simulink model "Simscape_model_Energy"  (R2026a)
settings: Solver=FixedStepAuto  StopTime=8  FixedStep=0.0001
model workspace (MATLAB code in the model file):
  | clear; clc; close all;
values from neighbouring files (symbols this model uses):
  black = partTemplate    [Parameters.m]    (also in Parameters_optimization.m = struct)
  blueBlock = partTemplate    [Parameters.m]    (also in Parameters_optimization.m = struct)
  cyan = partTemplate    [Parameters.m]    (also in Parameters_optimization.m = struct)
  g = 9.81    [Parameters.m]    (also in Parameters_optimization.m)
  greenBeam = partTemplate    [Parameters.m]    (also in Parameters_optimization.m = struct)
  greenBlock = partTemplate    [Parameters.m]    (also in Parameters_optimization.m = struct)
  grey = partTemplate    [Parameters.m]    (also in Parameters_optimization.m = struct)
  IMax = 16    [Parameters.m]    (also in Parameters_optimization.m)
  IMin = -16    [Parameters.m]    (also in Parameters_optimization.m)
  JM = 0.002    [Parameters.m]    (also in Parameters_optimization.m)
  KdA_pos = 1    [Parameters.m]    (also in Parameters_optimization.m = 5066.74)
  KdA_vel = 0    [Parameters.m]    (also in Parameters_optimization.m)
  KdB1_pos = 1    [Parameters.m]    (also in Parameters_optimization.m = 4.04669)
  KdB1_vel = 0    [Parameters.m]    (also in Parameters_optimization.m)
  KdB2_pos = 1    [Parameters.m]    (also in Parameters_optimization.m = 1.06194)
  KdB2_vel = 0    [Parameters.m]    (also in Parameters_optimization.m)
  KdG_pos = 1    [Parameters.m]    (also in Parameters_optimization.m = 1.01282)
  KdG_vel = 0    [Parameters.m]    (also in Parameters_optimization.m)
  KdH_pos = 1    [Parameters.m]    (also in Parameters_optimization.m = 16.6487)
  KdH_vel = 0    [Parameters.m]    (also in Parameters_optimization.m)
  KdI_pos = 1    [Parameters.m]    (also in Parameters_optimization.m = 2.31436)
  KdI_vel = 0    [Parameters.m]    (also in Parameters_optimization.m)
  KiA_pos = 2    [Parameters.m]    (also in Parameters_optimization.m = 1.00755)
  KiA_vel = 5    [Parameters.m]    (also in Parameters_optimization.m)
  KiB1_pos = 30    [Parameters.m]    (also in Parameters_optimization.m = 45.4381)
  KiB1_vel = 10    [Parameters.m]    (also in Parameters_optimization.m)
  KiB2_pos = 20    [Parameters.m]    (also in Parameters_optimization.m = 84.4311)
  KiB2_vel = 5    [Parameters.m]    (also in Parameters_optimization.m)
  KiG_pos = 30    [Parameters.m]    (also in Parameters_optimization.m = 81.5274)
  KiG_vel = 5    [Parameters.m]    (also in Parameters_optimization.m)
  KiH_pos = 10    [Parameters.m]    (also in Parameters_optimization.m = 20739.8)
  KiH_vel = 0    [Parameters.m]    (also in Parameters_optimization.m)
  KiI_pos = 0    [Parameters.m]    (also in Parameters_optimization.m = 1)
  KiI_vel = 0    [Parameters.m]    (also in Parameters_optimization.m)
  KmA = 1.5    [Parameters.m]    (also in Parameters_optimization.m = 1)
  KmB1 = 1.5    [Parameters.m]    (also in Parameters_optimization.m)
  KmB2 = 1.5    [Parameters.m]    (also in Parameters_optimization.m = 1)
  KmG = 0.5    [Parameters.m]    (also in Parameters_optimization.m)
  KmH = 1    [Parameters.m]    (also in Parameters_optimization.m = 0.5)
  KmI = 0.5    [Parameters.m]    (also in Parameters_optimization.m)
  KpA_pos = 150    [Parameters.m]    (also in Parameters_optimization.m = 1588.6)
  KpA_vel = 30    [Parameters.m]    (also in Parameters_optimization.m)
  KpB1_pos = 200    [Parameters.m]    (also in Parameters_optimization.m = 698393)
  KpB1_vel = 30    [Parameters.m]    (also in Parameters_optimization.m)
  KpB2_pos = 150    [Parameters.m]    (also in Parameters_optimization.m = 504375)
  KpB2_vel = 30    [Parameters.m]    (also in Parameters_optimization.m)
  KpG_pos = 100    [Parameters.m]    (also in Parameters_optimization.m = 2817.67)
  KpG_vel = 50    [Parameters.m]    (also in Parameters_optimization.m)
  KpH_pos = 100    [Parameters.m]    (also in Parameters_optimization.m = 12634.3)
  KpH_vel = 20    [Parameters.m]    (also in Parameters_optimization.m)
  KpI_pos = 50    [Parameters.m]    (also in Parameters_optimization.m = 2283.96)
  KpI_vel = 20    [Parameters.m]    (also in Parameters_optimization.m)
  LB1 = 0.8    [Parameters.m]    (also in Parameters_optimization.m)
  LB2 = 0.3    [Parameters.m]    (also in Parameters_optimization.m)
  LB3 = 0.24    [Parameters.m]    (also in Parameters_optimization.m)
  Lblack1 = 0.2    [Parameters.m]    (also in Parameters_optimization.m)
  LC1 = 0.4    [Parameters.m]    (also in Parameters_optimization.m)
  LC2 = 0.225    [Parameters.m]    (also in Parameters_optimization.m)
  LG1 = 0.3    [Parameters.m]    (also in Parameters_optimization.m)
  LG2 = 0.8    [Parameters.m]    (also in Parameters_optimization.m)
  Lgrey1 = 1.175    [Parameters.m]    (also in Parameters_optimization.m)
  lightBlue = partTemplate    [Parameters.m]    (also in Parameters_optimization.m = struct)
  LLB1 = 0.248    [Parameters.m]    (also in Parameters_optimization.m)
  LLB2 = 0.235    [Parameters.m]    (also in Parameters_optimization.m)
  LR1 = 1.05    [Parameters.m]    (also in Parameters_optimization.m)
  LW1 = 1.05    [Parameters.m]    (also in Parameters_optimization.m)
  nA = 200    [Parameters.m]    (also in Parameters_optimization.m = 100)
  nB1 = 200    [Parameters.m]    (also in Parameters_optimization.m = 100)
  nB2 = 200    [Parameters.m]    (also in Parameters_optimization.m)
  nG = 20    [Parameters.m]    (also in Parameters_optimization.m)
  nH = 100    [Parameters.m]    (also in Parameters_optimization.m = 50)
  nI = 20    [Parameters.m]    (also in Parameters_optimization.m)
  omegaFilterA_pos = 60    [Parameters.m]    (also in Parameters_optimization.m)
  omegaFilterA_vel = 60    [Parameters.m]    (also in Parameters_optimization.m)
  omegaFilterB1_pos = 60    [Parameters.m]    (also in Parameters_optimization.m)
  omegaFilterB1_vel = 60    [Parameters.m]    (also in Parameters_optimization.m)
  omegaFilterB2_pos = 60    [Parameters.m]    (also in Parameters_optimization.m)
  omegaFilterB2_vel = 60    [Parameters.m]    (also in Parameters_optimization.m)
  omegaFilterG_pos = 60    [Parameters.m]    (also in Parameters_optimization.m)
  omegaFilterG_vel = 60    [Parameters.m]    (also in Parameters_optimization.m)
  omegaFilterH_pos = 60    [Parameters.m]    (also in Parameters_optimization.m)
  omegaFilterH_vel = 60    [Parameters.m]    (also in Parameters_optimization.m)
  omegaFilterI_pos = 60    [Parameters.m]    (also in Parameters_optimization.m)
  omegaFilterI_vel = 60    [Parameters.m]    (also in Parameters_optimization.m)
  red = partTemplate    [Parameters.m]    (also in Parameters_optimization.m = struct)
  trajCoeff = coeff    [Parameters.m]    (also in Parameters_optimization.m = [2000 500 1600; Path_Planning_Robot.m)
  trajTime = t    [Parameters.m]    (also in Parameters_optimization.m = [0 2 4 6 8]; Path_Planning_Robot.m)
  w = 0.1    [Parameters.m]    (also in Parameters_optimization.m)
  white = partTemplate    [Parameters.m]    (also in Parameters_optimization.m = struct)
undefined symbols (not defined in the file or in its folder): X, Y, Z
libraries: sm_lib x102, nesl_utility x58, simulink x1
(part 2 of 4)

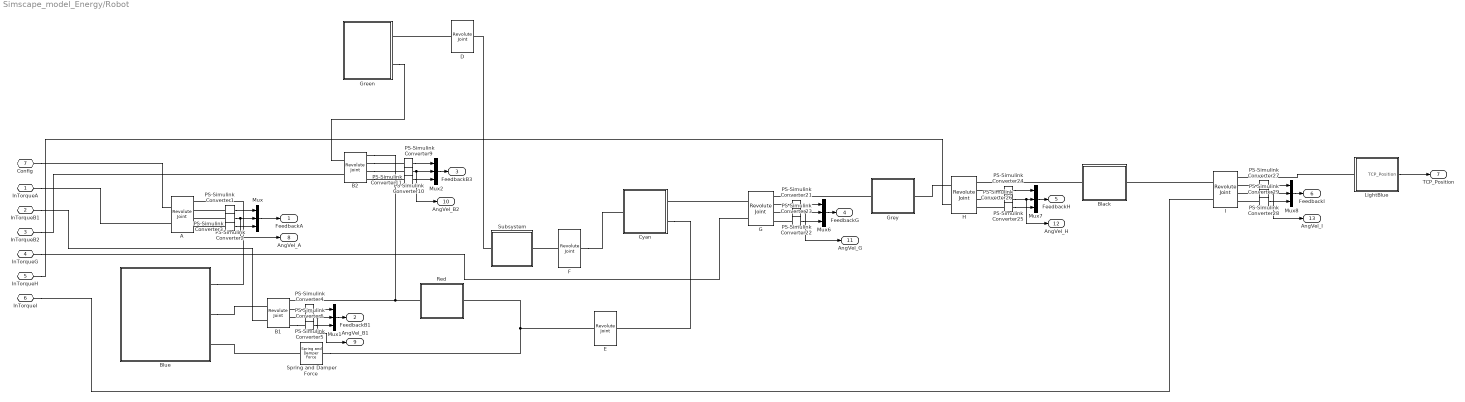
== system Simscape_model_Energy/Robot ==
  A : sm_lib/Joints/Revolute Joint  JointMode=Normal  CompositeWrenchDir=FollowerOnBase  CompositeWrenchFrame=BaseFrame  SenseConstraintForce=off  SenseConstraintTorque=off  SenseTotalForce=off  SenseTotalTorque=off  PositionTargetSpecify=on  PositionTargetPriority=High  PositionTargetValue=A0  PositionTargetValueUnits=rad  VelocityTargetSpecify=off  VelocityTargetPriority=High  VelocityTargetValue=0  VelocityTargetValueUnits=deg/s  EquilibriumPosition=0  EquilibriumPositionUnits=deg  SpringStiffness=0  SpringStiffnessUnits=N*m/deg  DampingCoefficient=0  DampingCoefficientUnits=N*m/(deg/s)  LowerLimitSpecify=off  LowerLimitBound=-90  LowerLimitBoundUnits=deg  LowerLimitStiffness=1e4  LowerLimitStiffnessUnits=N*m/deg  LowerLimitDamping=10  LowerLimitDampingUnits=N*m/(deg/s)  LowerLimitTransitionRegionWidth=0.1  LowerLimitTransitionRegionWidthUnits=deg  UpperLimitSpecify=off  UpperLimitBound=90  UpperLimitBoundUnits=deg  UpperLimitStiffness=1e4  UpperLimitStiffnessUnits=N*m/deg  UpperLimitDamping=10  UpperLimitDampingUnits=N*m/(deg/s)  UpperLimitTransitionRegionWidth=0.1  UpperLimitTransitionRegionWidthUnits=deg  TorqueActuationMode=InputTorque  MotionActuationMode=ComputedMotion  SensePosition=on  SenseVelocity=on  SenseAcceleration=on  SenseTorqueForce=off  SenseLowerLimitTorqueForce=off  SenseUpperLimitTorqueForce=off
  B1 : sm_lib/Joints/Revolute Joint  JointMode=Normal  CompositeWrenchDir=FollowerOnBase  CompositeWrenchFrame=BaseFrame  SenseConstraintForce=off  SenseConstraintTorque=off  SenseTotalForce=off  SenseTotalTorque=off  PositionTargetSpecify=on  PositionTargetPriority=High  PositionTargetValue=B10  PositionTargetValueUnits=rad  VelocityTargetSpecify=off  VelocityTargetPriority=High  VelocityTargetValue=0  VelocityTargetValueUnits=deg/s  EquilibriumPosition=0  EquilibriumPositionUnits=deg  SpringStiffness=0  SpringStiffnessUnits=N*m/deg  DampingCoefficient=0  DampingCoefficientUnits=N*m/(deg/s)  LowerLimitSpecify=on  LowerLimitBound=-80  LowerLimitBoundUnits=deg  LowerLimitStiffness=1e6  LowerLimitStiffnessUnits=N*m/deg  LowerLimitDamping=1000  LowerLimitDampingUnits=N*m/(deg/s)  LowerLimitTransitionRegionWidth=0.1  LowerLimitTransitionRegionWidthUnits=deg  UpperLimitSpecify=on  UpperLimitBound=80  UpperLimitBoundUnits=deg  UpperLimitStiffness=1e6  UpperLimitStiffnessUnits=N*m/deg  UpperLimitDamping=1000  UpperLimitDampingUnits=N*m/(deg/s)  UpperLimitTransitionRegionWidth=0.1  UpperLimitTransitionRegionWidthUnits=deg  TorqueActuationMode=InputTorque  MotionActuationMode=ComputedMotion  SensePosition=on  SenseVelocity=on  SenseAcceleration=on  SenseTorqueForce=off  SenseLowerLimitTorqueForce=off  SenseUpperLimitTorqueForce=off
  B2 : sm_lib/Joints/Revolute Joint  JointMode=Normal  CompositeWrenchDir=FollowerOnBase  CompositeWrenchFrame=BaseFrame  SenseConstraintForce=off  SenseConstraintTorque=off  SenseTotalForce=off  SenseTotalTorque=off  PositionTargetSpecify=on  PositionTargetPriority=High  PositionTargetValue=B20  PositionTargetValueUnits=rad  VelocityTargetSpecify=off  VelocityTargetPriority=High  VelocityTargetValue=0  VelocityTargetValueUnits=deg/s  EquilibriumPosition=0  EquilibriumPositionUnits=deg  SpringStiffness=0  SpringStiffnessUnits=N*m/deg  DampingCoefficient=0  DampingCoefficientUnits=N*m/(deg/s)  LowerLimitSpecify=off  LowerLimitBound=-90  LowerLimitBoundUnits=deg  LowerLimitStiffness=1e4  LowerLimitStiffnessUnits=N*m/deg  LowerLimitDamping=10  LowerLimitDampingUnits=N*m/(deg/s)  LowerLimitTransitionRegionWidth=0.1  LowerLimitTransitionRegionWidthUnits=deg  UpperLimitSpecify=off  UpperLimitBound=90  UpperLimitBoundUnits=deg  UpperLimitStiffness=1e4  UpperLimitStiffnessUnits=N*m/deg  UpperLimitDamping=10  UpperLimitDampingUnits=N*m/(deg/s)  UpperLimitTransitionRegionWidth=0.1  UpperLimitTransitionRegionWidthUnits=deg  TorqueActuationMode=InputTorque  MotionActuationMode=ComputedMotion  SensePosition=on  SenseVelocity=on  SenseAcceleration=on  SenseTorqueForce=off  SenseLowerLimitTorqueForce=off  SenseUpperLimitTorqueForce=off
  Black : Subsystem
  Blue : Subsystem
  Cyan : Subsystem
  D : sm_lib/Joints/Revolute Joint  JointMode=Normal  CompositeWrenchDir=FollowerOnBase  CompositeWrenchFrame=BaseFrame  SenseConstraintForce=off  SenseConstraintTorque=off  SenseTotalForce=off  SenseTotalTorque=off  PositionTargetSpecify=off  PositionTargetPriority=High  PositionTargetValue=0  PositionTargetValueUnits=deg  VelocityTargetSpecify=off  VelocityTargetPriority=High  VelocityTargetValue=0  VelocityTargetValueUnits=deg/s  EquilibriumPosition=0  EquilibriumPositionUnits=deg  SpringStiffness=0  SpringStiffnessUnits=N*m/deg  DampingCoefficient=0  DampingCoefficientUnits=N*m/(deg/s)  LowerLimitSpecify=off  LowerLimitBound=-90  LowerLimitBoundUnits=deg  LowerLimitStiffness=1e4  LowerLimitStiffnessUnits=N*m/deg  LowerLimitDamping=10  LowerLimitDampingUnits=N*m/(deg/s)  LowerLimitTransitionRegionWidth=0.1  LowerLimitTransitionRegionWidthUnits=deg  UpperLimitSpecify=off  UpperLimitBound=90  UpperLimitBoundUnits=deg  UpperLimitStiffness=1e4  UpperLimitStiffnessUnits=N*m/deg  UpperLimitDamping=10  UpperLimitDampingUnits=N*m/(deg/s)  UpperLimitTransitionRegionWidth=0.1  UpperLimitTransitionRegionWidthUnits=deg  TorqueActuationMode=NoTorque  MotionActuationMode=ComputedMotion  SensePosition=off  SenseVelocity=off  SenseAcceleration=off  SenseTorqueForce=off  SenseLowerLimitTorqueForce=off  SenseUpperLimitTorqueForce=off
  E : sm_lib/Joints/Revolute Joint  JointMode=Normal  CompositeWrenchDir=FollowerOnBase  CompositeWrenchFrame=BaseFrame  SenseConstraintForce=off  SenseConstraintTorque=off  SenseTotalForce=off  SenseTotalTorque=off  PositionTargetSpecify=off  PositionTargetPriority=High  PositionTargetValue=0  PositionTargetValueUnits=deg  VelocityTargetSpecify=off  VelocityTargetPriority=High  VelocityTargetValue=0  VelocityTargetValueUnits=deg/s  EquilibriumPosition=0  EquilibriumPositionUnits=deg  SpringStiffness=0  SpringStiffnessUnits=N*m/deg  DampingCoefficient=0  DampingCoefficientUnits=N*m/(deg/s)  LowerLimitSpecify=on  LowerLimitBound=-80  LowerLimitBoundUnits=deg  LowerLimitStiffness=1e6  LowerLimitStiffnessUnits=N*m/deg  LowerLimitDamping=100000  LowerLimitDampingUnits=N*m/(deg/s)  LowerLimitTransitionRegionWidth=0.1  LowerLimitTransitionRegionWidthUnits=deg  UpperLimitSpecify=on  UpperLimitBound=80  UpperLimitBoundUnits=deg  UpperLimitStiffness=1e6  UpperLimitStiffnessUnits=N*m/deg  UpperLimitDamping=100000  UpperLimitDampingUnits=N*m/(deg/s)  UpperLimitTransitionRegionWidth=0.1  UpperLimitTransitionRegionWidthUnits=deg  TorqueActuationMode=NoTorque  MotionActuationMode=ComputedMotion  SensePosition=off  SenseVelocity=off  SenseAcceleration=off  SenseTorqueForce=off  SenseLowerLimitTorqueForce=off  SenseUpperLimitTorqueForce=off
  F : sm_lib/Joints/Revolute Joint  JointMode=Normal  CompositeWrenchDir=FollowerOnBase  CompositeWrenchFrame=BaseFrame  SenseConstraintForce=off  SenseConstraintTorque=off  SenseTotalForce=off  SenseTotalTorque=off  PositionTargetSpecify=off  PositionTargetPriority=High  PositionTargetValue=0  PositionTargetValueUnits=deg  VelocityTargetSpecify=off  VelocityTargetPriority=High  VelocityTargetValue=0  VelocityTargetValueUnits=deg/s  EquilibriumPosition=0  EquilibriumPositionUnits=deg  SpringStiffness=0  SpringStiffnessUnits=N*m/deg  DampingCoefficient=0  DampingCoefficientUnits=N*m/(deg/s)  LowerLimitSpecify=off  LowerLimitBound=-90  LowerLimitBoundUnits=deg  LowerLimitStiffness=1e4  LowerLimitStiffnessUnits=N*m/deg  LowerLimitDamping=10  LowerLimitDampingUnits=N*m/(deg/s)  LowerLimitTransitionRegionWidth=0.1  LowerLimitTransitionRegionWidthUnits=deg  UpperLimitSpecify=off  UpperLimitBound=90  UpperLimitBoundUnits=deg  UpperLimitStiffness=1e4  UpperLimitStiffnessUnits=N*m/deg  UpperLimitDamping=10  UpperLimitDampingUnits=N*m/(deg/s)  UpperLimitTransitionRegionWidth=0.1  UpperLimitTransitionRegionWidthUnits=deg  TorqueActuationMode=NoTorque  MotionActuationMode=ComputedMotion  SensePosition=off  SenseVelocity=off  SenseAcceleration=off  SenseTorqueForce=off  SenseLowerLimitTorqueForce=off  SenseUpperLimitTorqueForce=off
  G : sm_lib/Joints/Revolute Joint  JointMode=Normal  CompositeWrenchDir=FollowerOnBase  CompositeWrenchFrame=BaseFrame  SenseConstraintForce=off  SenseConstraintTorque=off  SenseTotalForce=off  SenseTotalTorque=off  PositionTargetSpecify=on  PositionTargetPriority=High  PositionTargetValue=G0  PositionTargetValueUnits=rad  VelocityTargetSpecify=off  VelocityTargetPriority=High  VelocityTargetValue=0  VelocityTargetValueUnits=deg/s  EquilibriumPosition=0  EquilibriumPositionUnits=deg  SpringStiffness=0  SpringStiffnessUnits=N*m/deg  DampingCoefficient=0  DampingCoefficientUnits=N*m/(deg/s)  LowerLimitSpecify=off  LowerLimitBound=-90  LowerLimitBoundUnits=deg  LowerLimitStiffness=1e4  LowerLimitStiffnessUnits=N*m/deg  LowerLimitDamping=10  LowerLimitDampingUnits=N*m/(deg/s)  LowerLimitTransitionRegionWidth=0.1  LowerLimitTransitionRegionWidthUnits=deg  UpperLimitSpecify=off  UpperLimitBound=90  UpperLimitBoundUnits=deg  UpperLimitStiffness=1e4  UpperLimitStiffnessUnits=N*m/deg  UpperLimitDamping=10  UpperLimitDampingUnits=N*m/(deg/s)  UpperLimitTransitionRegionWidth=0.1  UpperLimitTransitionRegionWidthUnits=deg  TorqueActuationMode=InputTorque  MotionActuationMode=ComputedMotion  SensePosition=on  SenseVelocity=on  SenseAcceleration=on  SenseTorqueForce=off  SenseLowerLimitTorqueForce=off  SenseUpperLimitTorqueForce=off
  Green : Subsystem
  Grey : Subsystem
  H : sm_lib/Joints/Revolute Joint  JointMode=Normal  CompositeWrenchDir=FollowerOnBase  CompositeWrenchFrame=BaseFrame  SenseConstraintForce=off  SenseConstraintTorque=off  SenseTotalForce=off  SenseTotalTorque=off  PositionTargetSpecify=on  PositionTargetPriority=High  PositionTargetValue=H0  PositionTargetValueUnits=rad  VelocityTargetSpecify=off  VelocityTargetPriority=High  VelocityTargetValue=0  VelocityTargetValueUnits=deg/s  EquilibriumPosition=0  EquilibriumPositionUnits=deg  SpringStiffness=0  SpringStiffnessUnits=N*m/deg  DampingCoefficient=0  DampingCoefficientUnits=N*m/(deg/s)  LowerLimitSpecify=on  LowerLimitBound=-90  LowerLimitBoundUnits=deg  LowerLimitStiffness=1e4  LowerLimitStiffnessUnits=N*m/deg  LowerLimitDamping=10  LowerLimitDampingUnits=N*m/(deg/s)  LowerLimitTransitionRegionWidth=0.1  LowerLimitTransitionRegionWidthUnits=deg  UpperLimitSpecify=on  UpperLimitBound=90  UpperLimitBoundUnits=deg  UpperLimitStiffness=1e4  UpperLimitStiffnessUnits=N*m/deg  UpperLimitDamping=10  UpperLimitDampingUnits=N*m/(deg/s)  UpperLimitTransitionRegionWidth=0.1  UpperLimitTransitionRegionWidthUnits=deg  TorqueActuationMode=InputTorque  MotionActuationMode=ComputedMotion  SensePosition=on  SenseVelocity=on  SenseAcceleration=on  SenseTorqueForce=off  SenseLowerLimitTorqueForce=off  SenseUpperLimitTorqueForce=off
  I : sm_lib/Joints/Revolute Joint  JointMode=Normal  CompositeWrenchDir=FollowerOnBase  CompositeWrenchFrame=BaseFrame  SenseConstraintForce=off  SenseConstraintTorque=off  SenseTotalForce=off  SenseTotalTorque=off  PositionTargetSpecify=on  PositionTargetPriority=High  PositionTargetValue=I0  PositionTargetValueUnits=rad  VelocityTargetSpecify=off  VelocityTargetPriority=High  VelocityTargetValue=0  VelocityTargetValueUnits=deg/s  EquilibriumPosition=0  EquilibriumPositionUnits=deg  SpringStiffness=0  SpringStiffnessUnits=N*m/deg  DampingCoefficient=0  DampingCoefficientUnits=N*m/(deg/s)  LowerLimitSpecify=off  LowerLimitBound=-90  LowerLimitBoundUnits=deg  LowerLimitStiffness=1e4  LowerLimitStiffnessUnits=N*m/deg  LowerLimitDamping=10  LowerLimitDampingUnits=N*m/(deg/s)  LowerLimitTransitionRegionWidth=0.1  LowerLimitTransitionRegionWidthUnits=deg  UpperLimitSpecify=off  UpperLimitBound=90  UpperLimitBoundUnits=deg  UpperLimitStiffness=1e4  UpperLimitStiffnessUnits=N*m/deg  UpperLimitDamping=10  UpperLimitDampingUnits=N*m/(deg/s)  UpperLimitTransitionRegionWidth=0.1  UpperLimitTransitionRegionWidthUnits=deg  TorqueActuationMode=InputTorque  MotionActuationMode=ComputedMotion  SensePosition=on  SenseVelocity=on  SenseAcceleration=on  SenseTorqueForce=off  SenseLowerLimitTorqueForce=off  SenseUpperLimitTorqueForce=off
  LightBlue : Subsystem
  Mux{,1..2,6..8} (6 alike) : Mux  Inputs=3
  PS-Simulink Converter{1..6,9..11,21..29} (18 alike) : nesl_utility/PS-Simulink Converter  PhysicalDomain=network_engine_domain  SubClassName=ps_output  LeftPortType=input  RightPortType=output  PseudoPeriodic=off  Frequencies=[]  VectorFormat=inherit  Unit=inherit  AffineConversion=off
  Red : Subsystem
  Spring and Damper Force : sm_lib/Forces and Torques/Spring and Damper Force  NaturalLength=L0_spring  NaturalLengthUnits=m  SpringStiffness=k_spring  SpringStiffnessUnits=N/m  DampingCoefficient=0  DampingCoefficientUnits=N/(m/s)  SenseForce=off
  Subsystem : Subsystem
  InTorqueA : PMIOPort  Side=Left
  InTorqueB1 : PMIOPort  Port=2  Side=Left
  InTorqueB2 : PMIOPort  Port=3  Side=Left
  InTorqueG : PMIOPort  Port=4  Side=Left
  InTorqueH : PMIOPort  Port=5  Side=Left
  InTorqueI : PMIOPort  Port=6  Side=Left
  Config : PMIOPort  Port=7  Side=Left
  FeedbackA : Outport
  FeedbackB1 : Outport  Port=2
  FeedbackB3 : Outport  Port=3
  FeedbackG : Outport  Port=4
  FeedbackH : Outport  Port=5
  FeedbackI : Outport  Port=6
  TCP_Position : Outport  Port=7
  AngVel_A : Outport  Port=8
  AngVel_B1 : Outport  Port=9
  AngVel_B2 : Outport  Port=10
  AngVel_G : Outport  Port=11
  AngVel_H : Outport  Port=12
  AngVel_I : Outport  Port=13
  wires:
  PS-Simulink Converter6/1 -> Mux1/3
  PS-Simulink Converter5/1 -> AngVel_B1/1, Mux1/2
  PS-Simulink Converter28/1 -> AngVel_I/1, Mux8/2
  PS-Simulink Converter25/1 -> AngVel_H/1, Mux7/2
  PS-Simulink Converter9/1 -> Mux2/1
  PS-Simulink Converter26/1 -> Mux7/3
  PS-Simulink Converter27/1 -> Mux8/1
  PS-Simulink Converter24/1 -> Mux7/1
  PS-Simulink Converter2/1 -> AngVel_A/1, Mux/2
  PS-Simulink Converter22/1 -> AngVel_G/1, Mux6/2
  PS-Simulink Converter10/1 -> AngVel_B2/1, Mux2/2
  PS-Simulink Converter3/1 -> Mux/3
  PS-Simulink Converter11/1 -> Mux2/3
  Mux/1 -> FeedbackA/1
  PS-Simulink Converter1/1 -> Mux/1
  PS-Simulink Converter4/1 -> Mux1/1
  PS-Simulink Converter29/1 -> Mux8/3
  PS-Simulink Converter21/1 -> Mux6/1
  PS-Simulink Converter23/1 -> Mux6/3
  Mux8/1 -> FeedbackI/1
  Mux1/1 -> FeedbackB1/1
  Mux7/1 -> FeedbackH/1
  Mux6/1 -> FeedbackG/1
  Mux2/1 -> FeedbackB3/1
  LightBlue/1(TCP_Position) -> TCP_Position/1
  connections:
  B2/RConn1 -- Red/RConn1 -- B1/RConn1
  PS-Simulink Converter23/LConn1 -- G/RConn4
  LightBlue/LConn1 -- I/RConn1
  G/LConn1 -- Cyan/RConn1
  Spring and Damper Force/RConn1 -- E/LConn1 -- Red/LConn1
  PS-Simulink Converter25/LConn1 -- H/RConn3
  PS-Simulink Converter5/LConn1 -- B1/RConn3
  B2/RConn3 -- PS-Simulink Converter10/LConn1
  Black/LConn1 -- H/RConn1
  F/LConn1 -- Subsystem/LConn1
  Spring and Damper Force/LConn1 -- Blue/RConn3
  PS-Simulink Converter29/LConn1 -- I/RConn4
  Subsystem/RConn1 -- D/RConn1
  Green/RConn2 -- B2/LConn1
  I/LConn1 -- Black/RConn1
  B1/RConn4 -- PS-Simulink Converter6/LConn1
  PS-Simulink Converter2/LConn1 -- A/RConn3
  Blue/RConn2 -- B1/LConn1
  PS-Simulink Converter1/LConn1 -- A/RConn2
  PS-Simulink Converter27/LConn1 -- I/RConn2
  H/LConn1 -- Grey/RConn1
  PS-Simulink Converter3/LConn1 -- A/RConn4
  PS-Simulink Converter26/LConn1 -- H/RConn4
  PS-Simulink Converter22/LConn1 -- G/RConn3
  F/RConn1 -- Cyan/LConn1
  D/LConn1 -- Green/RConn1
  B2/RConn4 -- PS-Simulink Converter11/LConn1
  Grey/LConn1 -- G/RConn1
  Blue/RConn1 -- A/RConn1
  Cyan/RConn2 -- E/RConn1
  PS-Simulink Converter21/LConn1 -- G/RConn2
  B2/RConn2 -- PS-Simulink Converter9/LConn1
  PS-Simulink Converter4/LConn1 -- B1/RConn2
  PS-Simulink Converter28/LConn1 -- I/RConn3
  PS-Simulink Converter24/LConn1 -- H/RConn2
  InTorqueA/RConn1 -- A/LConn2
  InTorqueB1/RConn1 -- B1/LConn2
  InTorqueB2/RConn1 -- B2/LConn2
  InTorqueG/RConn1 -- G/LConn2
  InTorqueH/RConn1 -- H/LConn2
  InTorqueI/RConn1 -- I/LConn2
  Config/RConn1 -- A/LConn1

== system Simscape_model_Energy/Subsystem ==
  torque : Inport
  angularVelocity : Inport  Port=2
  Integrator : Integrator
  Integrator1 : Integrator
  MATLAB Function7 : MATLAB Function  TreatAsAtomicUnit=on
  E_motoring_A : Outport
  E_generating_A : Outport  Port=2
  wires:
  Integrator/1 -> E_motoring_A/1  "E_motoring_A"
  torque/1 -> MATLAB Function7/1(torque)
  MATLAB Function7/1(P_motoring) -> Integrator/1
  angularVelocity/1 -> MATLAB Function7/2(angularVelocity)
  Integrator1/1 -> E_generating_A/1  "E_generating_A"
  MATLAB Function7/2(P_generating) -> Integrator1/1

== system Simscape_model_Energy/Subsystem1 ==
  torque : Inport
  angularVelocity : Inport  Port=2
  Integrator : Integrator
  Integrator1 : Integrator
  MATLAB Function7 : MATLAB Function  TreatAsAtomicUnit=on
  E_motoring_B1 : Outport
  E_generating_B1 : Outport  Port=2
  wires:
  Integrator/1 -> E_motoring_B1/1  "E_motoring_A"
  torque/1 -> MATLAB Function7/1(torque)
  MATLAB Function7/1(P_motoring) -> Integrator/1
  angularVelocity/1 -> MATLAB Function7/2(angularVelocity)
  Integrator1/1 -> E_generating_B1/1  "E_generating_A"
  MATLAB Function7/2(P_generating) -> Integrator1/1

== system Simscape_model_Energy/Subsystem2 ==
  torque : Inport
  angularVelocity : Inport  Port=2
  Integrator : Integrator
  Integrator1 : Integrator
  MATLAB Function7 : MATLAB Function  TreatAsAtomicUnit=on
  E_motoring_B2 : Outport
  E_generating_B2 : Outport  Port=2
  wires:
  Integrator/1 -> E_motoring_B2/1  "E_motoring_A"
  torque/1 -> MATLAB Function7/1(torque)
  MATLAB Function7/1(P_motoring) -> Integrator/1
  angularVelocity/1 -> MATLAB Function7/2(angularVelocity)
  Integrator1/1 -> E_generating_B2/1  "E_generating_A"
  MATLAB Function7/2(P_generating) -> Integrator1/1

== system Simscape_model_Energy/Subsystem3 ==
  torque : Inport
  angularVelocity : Inport  Port=2
  Integrator : Integrator
  Integrator1 : Integrator
  MATLAB Function7 : MATLAB Function  TreatAsAtomicUnit=on
  E_motoring_G : Outport
  E_generating_G : Outport  Port=2
  wires:
  Integrator/1 -> E_motoring_G/1  "E_motoring_A"
  torque/1 -> MATLAB Function7/1(torque)
  MATLAB Function7/1(P_motoring) -> Integrator/1
  angularVelocity/1 -> MATLAB Function7/2(angularVelocity)
  Integrator1/1 -> E_generating_G/1  "E_generating_A"
  MATLAB Function7/2(P_generating) -> Integrator1/1

== system Simscape_model_Energy/Subsystem4 ==
  torque : Inport
  angularVelocity : Inport  Port=2
  Integrator : Integrator
  Integrator1 : Integrator
  MATLAB Function7 : MATLAB Function  TreatAsAtomicUnit=on
  E_motoring_H : Outport
  E_generating_H : Outport  Port=2
  wires:
  Integrator/1 -> E_motoring_H/1  "E_motoring_A"
  torque/1 -> MATLAB Function7/1(torque)
  MATLAB Function7/1(P_motoring) -> Integrator/1
  angularVelocity/1 -> MATLAB Function7/2(angularVelocity)
  Integrator1/1 -> E_generating_H/1  "E_generating_A"
  MATLAB Function7/2(P_generating) -> Integrator1/1

== system Simscape_model_Energy/Subsystem5 ==
  torque : Inport
  angularVelocity : Inport  Port=2
  Integrator : Integrator
  Integrator1 : Integrator
  MATLAB Function7 : MATLAB Function  TreatAsAtomicUnit=on
  E_motoring_I : Outport
  E_generating_I : Outport  Port=2
  wires:
  Integrator/1 -> E_motoring_I/1  "E_motoring_A"
  torque/1 -> MATLAB Function7/1(torque)
  MATLAB Function7/1(P_motoring) -> Integrator/1
  angularVelocity/1 -> MATLAB Function7/2(angularVelocity)
  Integrator1/1 -> E_generating_I/1  "E_generating_A"
  MATLAB Function7/2(P_generating) -> Integrator1/1

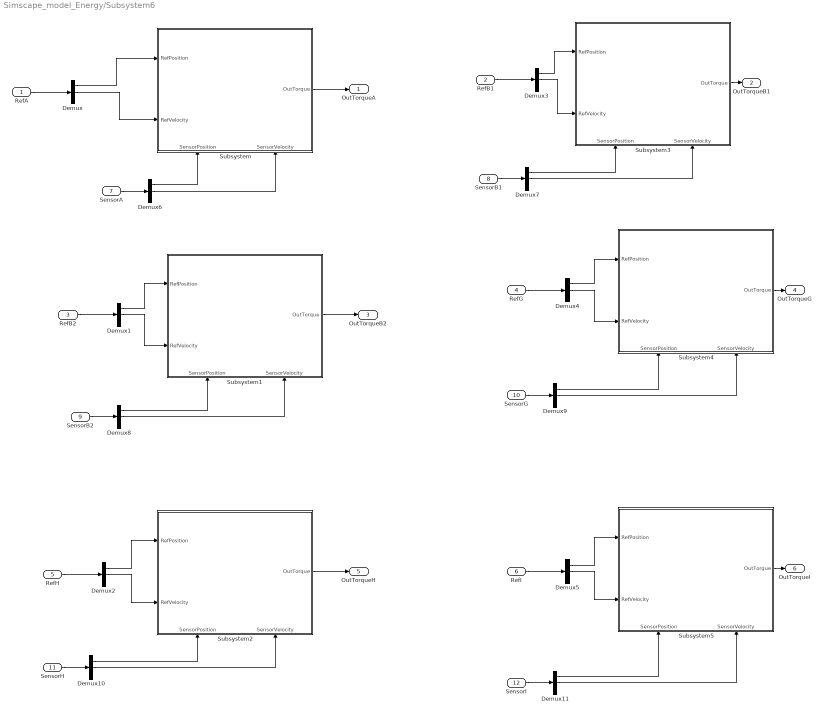
== system Simscape_model_Energy/Subsystem6 ==
  RefA : Inport
  RefB1 : Inport  Port=2
  RefB2 : Inport  Port=3
  RefG : Inport  Port=4
  RefH : Inport  Port=5
  RefI : Inport  Port=6
  SensorA : Inport  Port=7
  SensorB1 : Inport  Port=8
  SensorB2 : Inport  Port=9
  SensorG : Inport  Port=10
  SensorH : Inport  Port=11
  SensorI : Inport  Port=12
  Demux{,1..11} (12 alike) : Demux  Outputs=3
  Subsystem : Subsystem
      settings: PortSchema="{\"entries\":[{\"content\":{\"sides\":[{\"content\":{\"connectorIds\":[\"In1\",\"In2\"]},\"type\":\"ConnectorPlacement.EquallySpacedRectSide\",\"uuid\":\"51550f40-279e-4723-9a78-98dcf3f698a2\"},{\"content\":{\"connectorIds\":[\"Out1\"],\"side\":\"RIGHT\"},\"type\":\"ConnectorPlacement.EquallySpacedRectSide\",\"uuid\":\"f243d76f-4e9d-407e-a230-76bea4453255\"},{\"content\":{\"side\":\"TOP\"},\"type\":\"ConnectorPlacement.EquallySpacedRectSide\",\"uuid\":\"5b6b6dd7-8a33-494a-8ee5-fc7698c2bf83\"},{\"content\":{\"connectorIds\":[\"In3\",\"In4\"],\"side\":\"BOTTOM\"},\"type\":\"ConnectorPlacement.EquallySpacedRectSide\",\"uuid\":\"d720744c-358d-4588-a5fe-fa324fd98b41\"}]},\"type\":\"ConnectorPlacement.EquallySpacedConnector\",\"uuid\":\"b5ef8a6e-2b84-4a51-bcfc-62a4469380e6\"}],\"packageUris\":[\"http://schema.mathworks.com/mf0/Connector/R2020b\"],\"version\":\"1.0\"}"
  Subsystem1 : Subsystem
      settings: PortSchema="{\"entries\":[{\"content\":{\"sides\":[{\"content\":{\"connectorIds\":[\"In1\",\"In2\"]},\"type\":\"ConnectorPlacement.EquallySpacedRectSide\",\"uuid\":\"51550f40-279e-4723-9a78-98dcf3f698a2\"},{\"content\":{\"connectorIds\":[\"Out1\"],\"side\":\"RIGHT\"},\"type\":\"ConnectorPlacement.EquallySpacedRectSide\",\"uuid\":\"f243d76f-4e9d-407e-a230-76bea4453255\"},{\"content\":{\"side\":\"TOP\"},\"type\":\"ConnectorPlacement.EquallySpacedRectSide\",\"uuid\":\"5b6b6dd7-8a33-494a-8ee5-fc7698c2bf83\"},{\"content\":{\"connectorIds\":[\"In3\",\"In4\"],\"side\":\"BOTTOM\"},\"type\":\"ConnectorPlacement.EquallySpacedRectSide\",\"uuid\":\"d720744c-358d-4588-a5fe-fa324fd98b41\"}]},\"type\":\"ConnectorPlacement.EquallySpacedConnector\",\"uuid\":\"b5ef8a6e-2b84-4a51-bcfc-62a4469380e6\"}],\"packageUris\":[\"http://schema.mathworks.com/mf0/Connector/R2020b\"],\"version\":\"1.0\"}"
  Subsystem2 : Subsystem
      settings: PortSchema="{\"entries\":[{\"content\":{\"sides\":[{\"content\":{\"connectorIds\":[\"In1\",\"In2\"]},\"type\":\"ConnectorPlacement.EquallySpacedRectSide\",\"uuid\":\"51550f40-279e-4723-9a78-98dcf3f698a2\"},{\"content\":{\"connectorIds\":[\"Out1\"],\"side\":\"RIGHT\"},\"type\":\"ConnectorPlacement.EquallySpacedRectSide\",\"uuid\":\"f243d76f-4e9d-407e-a230-76bea4453255\"},{\"content\":{\"side\":\"TOP\"},\"type\":\"ConnectorPlacement.EquallySpacedRectSide\",\"uuid\":\"5b6b6dd7-8a33-494a-8ee5-fc7698c2bf83\"},{\"content\":{\"connectorIds\":[\"In3\",\"In4\"],\"side\":\"BOTTOM\"},\"type\":\"ConnectorPlacement.EquallySpacedRectSide\",\"uuid\":\"d720744c-358d-4588-a5fe-fa324fd98b41\"}]},\"type\":\"ConnectorPlacement.EquallySpacedConnector\",\"uuid\":\"b5ef8a6e-2b84-4a51-bcfc-62a4469380e6\"}],\"packageUris\":[\"http://schema.mathworks.com/mf0/Connector/R2020b\"],\"version\":\"1.0\"}"
  Subsystem3 : Subsystem
      settings: PortSchema="{\"entries\":[{\"content\":{\"sides\":[{\"content\":{\"connectorIds\":[\"In1\",\"In2\"]},\"type\":\"ConnectorPlacement.EquallySpacedRectSide\",\"uuid\":\"51550f40-279e-4723-9a78-98dcf3f698a2\"},{\"content\":{\"connectorIds\":[\"Out1\"],\"side\":\"RIGHT\"},\"type\":\"ConnectorPlacement.EquallySpacedRectSide\",\"uuid\":\"f243d76f-4e9d-407e-a230-76bea4453255\"},{\"content\":{\"side\":\"TOP\"},\"type\":\"ConnectorPlacement.EquallySpacedRectSide\",\"uuid\":\"5b6b6dd7-8a33-494a-8ee5-fc7698c2bf83\"},{\"content\":{\"connectorIds\":[\"In3\",\"In4\"],\"side\":\"BOTTOM\"},\"type\":\"ConnectorPlacement.EquallySpacedRectSide\",\"uuid\":\"d720744c-358d-4588-a5fe-fa324fd98b41\"}]},\"type\":\"ConnectorPlacement.EquallySpacedConnector\",\"uuid\":\"b5ef8a6e-2b84-4a51-bcfc-62a4469380e6\"}],\"packageUris\":[\"http://schema.mathworks.com/mf0/Connector/R2020b\"],\"version\":\"1.0\"}"
  Subsystem4 : Subsystem
      settings: PortSchema="{\"entries\":[{\"content\":{\"sides\":[{\"content\":{\"connectorIds\":[\"In1\",\"In2\"]},\"type\":\"ConnectorPlacement.EquallySpacedRectSide\",\"uuid\":\"51550f40-279e-4723-9a78-98dcf3f698a2\"},{\"content\":{\"connectorIds\":[\"Out1\"],\"side\":\"RIGHT\"},\"type\":\"ConnectorPlacement.EquallySpacedRectSide\",\"uuid\":\"f243d76f-4e9d-407e-a230-76bea4453255\"},{\"content\":{\"side\":\"TOP\"},\"type\":\"ConnectorPlacement.EquallySpacedRectSide\",\"uuid\":\"5b6b6dd7-8a33-494a-8ee5-fc7698c2bf83\"},{\"content\":{\"connectorIds\":[\"In3\",\"In4\"],\"side\":\"BOTTOM\"},\"type\":\"ConnectorPlacement.EquallySpacedRectSide\",\"uuid\":\"d720744c-358d-4588-a5fe-fa324fd98b41\"}]},\"type\":\"ConnectorPlacement.EquallySpacedConnector\",\"uuid\":\"b5ef8a6e-2b84-4a51-bcfc-62a4469380e6\"}],\"packageUris\":[\"http://schema.mathworks.com/mf0/Connector/R2020b\"],\"version\":\"1.0\"}"
  Subsystem5 : Subsystem
      settings: PortSchema="{\"entries\":[{\"content\":{\"sides\":[{\"content\":{\"connectorIds\":[\"In1\",\"In2\"]},\"type\":\"ConnectorPlacement.EquallySpacedRectSide\",\"uuid\":\"51550f40-279e-4723-9a78-98dcf3f698a2\"},{\"content\":{\"connectorIds\":[\"Out1\"],\"side\":\"RIGHT\"},\"type\":\"ConnectorPlacement.EquallySpacedRectSide\",\"uuid\":\"f243d76f-4e9d-407e-a230-76bea4453255\"},{\"content\":{\"side\":\"TOP\"},\"type\":\"ConnectorPlacement.EquallySpacedRectSide\",\"uuid\":\"5b6b6dd7-8a33-494a-8ee5-fc7698c2bf83\"},{\"content\":{\"connectorIds\":[\"In3\",\"In4\"],\"side\":\"BOTTOM\"},\"type\":\"ConnectorPlacement.EquallySpacedRectSide\",\"uuid\":\"d720744c-358d-4588-a5fe-fa324fd98b41\"}]},\"type\":\"ConnectorPlacement.EquallySpacedConnector\",\"uuid\":\"b5ef8a6e-2b84-4a51-bcfc-62a4469380e6\"}],\"packageUris\":[\"http://schema.mathworks.com/mf0/Connector/R2020b\"],\"version\":\"1.0\"}"
  OutTorqueA : Outport
  OutTorqueB1 : Outport  Port=2
  OutTorqueB2 : Outport  Port=3
  OutTorqueG : Outport  Port=4
  OutTorqueH : Outport  Port=5
  OutTorqueI : Outport  Port=6
  wires:
  Demux/2 -> Subsystem/2(RefVelocity)
  Demux/1 -> Subsystem/1(RefPosition)
  Subsystem2/1(OutTorque) -> OutTorqueH/1
  Subsystem3/1(OutTorque) -> OutTorqueB1/1
  Subsystem4/1(OutTorque) -> OutTorqueG/1
  Subsystem1/1(OutTorque) -> OutTorqueB2/1
  Subsystem/1(OutTorque) -> OutTorqueA/1
  Subsystem5/1(OutTorque) -> OutTorqueI/1
  RefA/1 -> Demux/1
  RefB2/1 -> Demux1/1
  Demux1/1 -> Subsystem1/1(RefPosition)
  Demux1/2 -> Subsystem1/2(RefVelocity)
  RefH/1 -> Demux2/1
  Demux2/1 -> Subsystem2/1(RefPosition)
  Demux2/2 -> Subsystem2/2(RefVelocity)
  RefB1/1 -> Demux3/1
  Demux3/1 -> Subsystem3/1(RefPosition)
  Demux3/2 -> Subsystem3/2(RefVelocity)
  RefG/1 -> Demux4/1
  Demux4/1 -> Subsystem4/1(RefPosition)
  Demux4/2 -> Subsystem4/2(RefVelocity)
  RefI/1 -> Demux5/1
  Demux5/1 -> Subsystem5/1(RefPosition)
  Demux5/2 -> Subsystem5/2(RefVelocity)
  SensorA/1 -> Demux6/1
  Demux6/1 -> Subsystem/3(SensorPosition)
  Demux6/2 -> Subsystem/4(SensorVelocity)
  SensorB1/1 -> Demux7/1
  Demux7/1 -> Subsystem3/3(SensorPosition)
  Demux7/2 -> Subsystem3/4(SensorVelocity)
  SensorB2/1 -> Demux8/1
  Demux8/1 -> Subsystem1/3(SensorPosition)
  Demux8/2 -> Subsystem1/4(SensorVelocity)
  SensorG/1 -> Demux9/1
  Demux9/1 -> Subsystem4/3(SensorPosition)
  Demux9/2 -> Subsystem4/4(SensorVelocity)
  SensorH/1 -> Demux10/1
  Demux10/1 -> Subsystem2/3(SensorPosition)
  Demux10/2 -> Subsystem2/4(SensorVelocity)
  SensorI/1 -> Demux11/1
  Demux11/1 -> Subsystem5/3(SensorPosition)
  Demux11/2 -> Subsystem5/4(SensorVelocity)

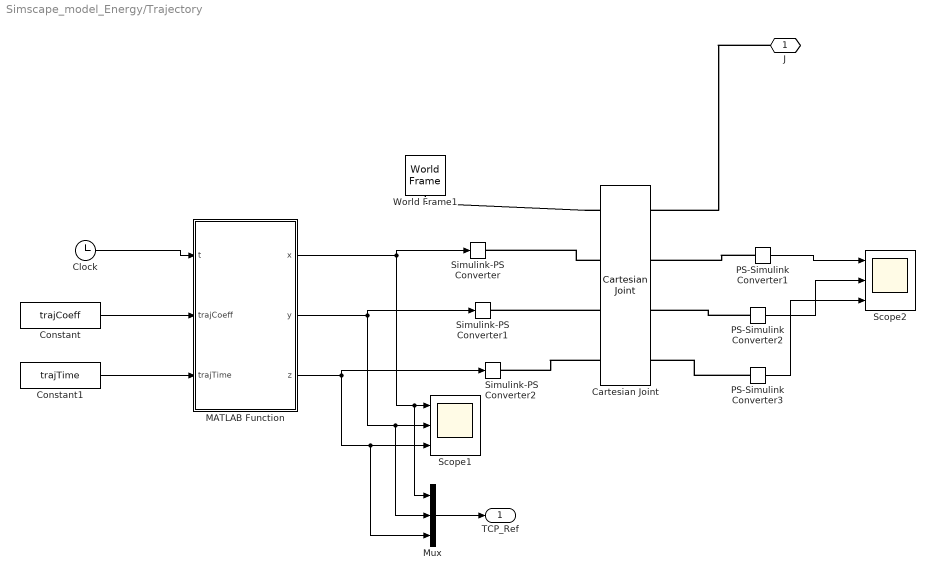
== system Simscape_model_Energy/Trajectory ==
  Cartesian Joint : sm_lib/Joints/Cartesian Joint  JointMode=Normal  CompositeWrenchDir=FollowerOnBase  CompositeWrenchFrame=BaseFrame  SenseConstraintForce=off  SenseConstraintTorque=off  SenseTotalForce=off  SenseTotalTorque=off  PxPositionTargetSpecify=off  PxPositionTargetPriority=High  PxPositionTargetValue=0  PxPositionTargetValueUnits=m  PxVelocityTargetSpecify=off  PxVelocityTargetPriority=High  PxVelocityTargetValue=0  PxVelocityTargetValueUnits=m/s  PxEquilibriumPosition=0  PxEquilibriumPositionUnits=m  PxSpringStiffness=0  PxSpringStiffnessUnits=N/m  PxDampingCoefficient=0  PxDampingCoefficientUnits=N/(m/s)  PxLowerLimitSpecify=off  PxLowerLimitBound=-1  PxLowerLimitBoundUnits=m  PxLowerLimitStiffness=1e6  PxLowerLimitStiffnessUnits=N/m  PxLowerLimitDamping=1e3  PxLowerLimitDampingUnits=N/(m/s)  PxLowerLimitTransitionRegionWidth=1e-4  PxLowerLimitTransitionRegionWidthUnits=m  PxUpperLimitSpecify=off  PxUpperLimitBound=1  PxUpperLimitBoundUnits=m  PxUpperLimitStiffness=1e6  PxUpperLimitStiffnessUnits=N/m  PxUpperLimitDamping=1e3  PxUpperLimitDampingUnits=N/(m/s)  PxUpperLimitTransitionRegionWidth=1e-4  PxUpperLimitTransitionRegionWidthUnits=m  PxTorqueActuationMode=ComputedTorque  PxMotionActuationMode=InputMotion  PxSensePosition=on  PxSenseVelocity=off  PxSenseAcceleration=off  PxSenseTorqueForce=off  PxSenseLowerLimitTorqueForce=off  PxSenseUpperLimitTorqueForce=off  PyPositionTargetSpecify=off  PyPositionTargetPriority=High  PyPositionTargetValue=0  PyPositionTargetValueUnits=m  PyVelocityTargetSpecify=off  PyVelocityTargetPriority=High  PyVelocityTargetValue=0  PyVelocityTargetValueUnits=m/s  PyEquilibriumPosition=0  PyEquilibriumPositionUnits=m  PySpringStiffness=0  PySpringStiffnessUnits=N/m  PyDampingCoefficient=0  PyDampingCoefficientUnits=N/(m/s)  PyLowerLimitSpecify=off  PyLowerLimitBound=-1  PyLowerLimitBoundUnits=m  PyLowerLimitStiffness=1e6  PyLowerLimitStiffnessUnits=N/m  PyLowerLimitDamping=1e3  PyLowerLimitDampingUnits=N/(m/s)  PyLowerLimitTransitionRegionWidth=1e-4  PyLowerLimitTransitionRegionWidthUnits=m  PyUpperLimitSpecify=off  PyUpperLimitBound=1  PyUpperLimitBoundUnits=m  PyUpperLimitStiffness=1e6  PyUpperLimitStiffnessUnits=N/m  PyUpperLimitDamping=1e3  PyUpperLimitDampingUnits=N/(m/s)  PyUpperLimitTransitionRegionWidth=1e-4  PyUpperLimitTransitionRegionWidthUnits=m  PyTorqueActuationMode=ComputedTorque  PyMotionActuationMode=InputMotion  PySensePosition=on  PySenseVelocity=off  PySenseAcceleration=off  PySenseTorqueForce=off  PySenseLowerLimitTorqueForce=off  PySenseUpperLimitTorqueForce=off  PzPositionTargetSpecify=off  PzPositionTargetPriority=High  PzPositionTargetValue=0  PzPositionTargetValueUnits=m  PzVelocityTargetSpecify=off  PzVelocityTargetPriority=High  PzVelocityTargetValue=0  PzVelocityTargetValueUnits=m/s  PzEquilibriumPosition=0  PzEquilibriumPositionUnits=m  PzSpringStiffness=0  PzSpringStiffnessUnits=N/m  PzDampingCoefficient=0  PzDampingCoefficientUnits=N/(m/s)  PzLowerLimitSpecify=off  PzLowerLimitBound=-1  PzLowerLimitBoundUnits=m  PzLowerLimitStiffness=1e6  PzLowerLimitStiffnessUnits=N/m  PzLowerLimitDamping=1e3  PzLowerLimitDampingUnits=N/(m/s)  PzLowerLimitTransitionRegionWidth=1e-4  PzLowerLimitTransitionRegionWidthUnits=m  PzUpperLimitSpecify=off  PzUpperLimitBound=1  PzUpperLimitBoundUnits=m  PzUpperLimitStiffness=1e6  PzUpperLimitStiffnessUnits=N/m  PzUpperLimitDamping=1e3  PzUpperLimitDampingUnits=N/(m/s)  PzUpperLimitTransitionRegionWidth=1e-4  PzUpperLimitTransitionRegionWidthUnits=m  PzTorqueActuationMode=ComputedTorque  PzMotionActuationMode=InputMotion  PzSensePosition=on  PzSenseVelocity=off  PzSenseAcceleration=off  PzSenseTorqueForce=off  PzSenseLowerLimitTorqueForce=off  PzSenseUpperLimitTorqueForce=off
  Clock : Clock
  Constant : Constant  Value=trajCoeff
  Constant1 : Constant  Value=trajTime
  MATLAB Function : MATLAB Function  TreatAsAtomicUnit=on
  Mux : Mux  Inputs=3
  PS-Simulink Converter1 : nesl_utility/PS-Simulink Converter  PhysicalDomain=network_engine_domain  SubClassName=ps_output  LeftPortType=input  RightPortType=output  PseudoPeriodic=off  Frequencies=[]  VectorFormat=inherit  Unit=inherit  AffineConversion=off
  PS-Simulink Converter2 : nesl_utility/PS-Simulink Converter  PhysicalDomain=network_engine_domain  SubClassName=ps_output  LeftPortType=input  RightPortType=output  PseudoPeriodic=off  Frequencies=[]  VectorFormat=inherit  Unit=inherit  AffineConversion=off
  PS-Simulink Converter3 : nesl_utility/PS-Simulink Converter  PhysicalDomain=network_engine_domain  SubClassName=ps_output  LeftPortType=input  RightPortType=output  PseudoPeriodic=off  Frequencies=[]  VectorFormat=inherit  Unit=inherit  AffineConversion=off
  Scope1 : Scope  NumInputPorts=3
      settings: ActiveDisplayYMinimum=-0.85197636389002107  ActiveDisplayYMaximum=2.3356362626544458
  Scope2 : Scope  NumInputPorts=3
      settings: ActiveDisplayYMinimum=-0.85197636389002107  ActiveDisplayYMaximum=2.3356362626544458  DataLoggingVariableName=ScopeData2
  Simulink-PS Converter : nesl_utility/Simulink-PS Converter  PhysicalDomain=network_engine_domain  SubClassName=ps_input  LeftPortType=input  RightPortType=output  PseudoPeriodic=off  Frequencies=[]  NoiseDistribution=none  NoiseParameters=[]  Unit=1  AffineConversion=off  FilteringAndDerivatives=filter  SimscapeFilterOrder=2  InputFilterTimeConstant=0.001  UdotUserProvided=0
  Simulink-PS Converter1 : nesl_utility/Simulink-PS Converter  PhysicalDomain=network_engine_domain  SubClassName=ps_input  LeftPortType=input  RightPortType=output  PseudoPeriodic=off  Frequencies=[]  NoiseDistribution=none  NoiseParameters=[]  Unit=1  AffineConversion=off  FilteringAndDerivatives=filter  SimscapeFilterOrder=2  InputFilterTimeConstant=0.001  UdotUserProvided=0
  Simulink-PS Converter2 : nesl_utility/Simulink-PS Converter  PhysicalDomain=network_engine_domain  SubClassName=ps_input  LeftPortType=input  RightPortType=output  PseudoPeriodic=off  Frequencies=[]  NoiseDistribution=none  NoiseParameters=[]  Unit=1  AffineConversion=off  FilteringAndDerivatives=filter  SimscapeFilterOrder=2  InputFilterTimeConstant=0.001  UdotUserProvided=0
  World Frame1 : sm_lib/Frames and Transforms/World Frame
  J : PMIOPort  Side=Right
  TCP_Ref : Outport
  wires:
  Constant/1 -> MATLAB Function/2(trajCoeff)
  MATLAB Function/2(y) -> Simulink-PS Converter1/1, Mux/2, Scope1/2
  MATLAB Function/3(z) -> Simulink-PS Converter2/1, Scope1/3, Mux/3
  PS-Simulink Converter2/1 -> Scope2/2
  PS-Simulink Converter3/1 -> Scope2/3
  MATLAB Function/1(x) -> Simulink-PS Converter/1, Mux/1, Scope1/1
  Clock/1 -> MATLAB Function/1(t)
  PS-Simulink Converter1/1 -> Scope2/1
  Constant1/1 -> MATLAB Function/3(trajTime)
  Mux/1 -> TCP_Ref/1
  connections:
  J/RConn1 -- Cartesian Joint/RConn1
  PS-Simulink Converter2/LConn1 -- Cartesian Joint/RConn3
  Cartesian Joint/LConn1 -- World Frame1/RConn1
  Cartesian Joint/LConn4 -- Simulink-PS Converter2/RConn1
  Cartesian Joint/LConn2 -- Simulink-PS Converter/RConn1
  Cartesian Joint/LConn3 -- Simulink-PS Converter1/RConn1
  PS-Simulink Converter1/LConn1 -- Cartesian Joint/RConn2
  PS-Simulink Converter3/LConn1 -- Cartesian Joint/RConn4

== system Simscape_model_Energy/ReferenceGenerator/Black ==
  Black : sm_lib/Body Elements/Brick Solid  BrickDimensions=[Lblack1 w w]  BrickDimensionsUnits=m  ExportEntireGeometry=off  InertiaType=Custom  BasedOnType=Density  Density=1000  DensityUnits=kg/m^3  Mass=black.m  MassUnits=kg  CenterOfMass=[0 0 0]  CenterOfMassUnits=m  MomentsOfInertia=[black.Ix black.Iy black.Iz]  MomentsOfInertiaUnits=kg*m^2  ProductsOfInertia=[0 0 0]  ProductsOfInertiaUnits=kg*m^2  GraphicType=FromGeometry  MarkerShape=Sphere  MarkerSize=10  GraphicVisPropType=SimpleVisualProperties  GraphicDiffuseColor=[0 0 0]  GraphicOpacity=1  GraphicSpecularColor=[0.5 0.5 0.5 1.0]  GraphicAmbientColor=[0.15 0.15 0.15 1.0]  GraphicEmissiveColor=[0.0 0.0 0.0 1.0]  GraphicShininess=75  DoExposeReferenceFrame=on  SerializedFrames=<Frames/>
  PlacIementI : sm_lib/Frames and Transforms/Rigid Transform  RotationMethod=RotationSequence  FollAlignAxisA=+X  BaseAlignAxisA=+Y  FollAlignAxisB=+Y  BaseAlignAxisB=+Z  RotationStandardAxis=+Z  RotationAngle=0  RotationAngleUnits=deg  RotationArbitraryAxis=[0 0 1]  RotationSequenceAxes=FollowerAxes  RotationSequence=XYX  RotationSequenceAngles=[0 90 0]  RotationSequenceAnglesUnits=deg  RotationMatrix=[1 0 0;0 1 0;0 0 1]  Quaternion=[1 0 0 0]  TranslationMethod=Cartesian  TranslationCartesianOffset=[Lblack1/2 0 0]  TranslationCartesianOffsetUnits=m  TranslationStandardAxis=+Z  TranslationStandardOffset=0  TranslationStandardOffsetUnits=m  TranslationROffset=0  TranslationROffsetUnits=m  TranslationThetaOffset=0  TranslationThetaOffsetUnits=deg  TranslationZOffset=0  TranslationZOffsetUnits=m
  PlacementBlack : sm_lib/Frames and Transforms/Rigid Transform  RotationMethod=None  FollAlignAxisA=+X  BaseAlignAxisA=+Y  FollAlignAxisB=+Y  BaseAlignAxisB=+Z  RotationStandardAxis=+Z  RotationAngle=0  RotationAngleUnits=deg  RotationArbitraryAxis=[0 0 1]  RotationSequenceAxes=FollowerAxes  RotationSequence=XYX  RotationSequenceAngles=[0 0 0]  RotationSequenceAnglesUnits=deg  RotationMatrix=[1 0 0;0 1 0;0 0 1]  Quaternion=[1 0 0 0]  TranslationMethod=Cartesian  TranslationCartesianOffset=[Lblack1/2 0 0]  TranslationCartesianOffsetUnits=m  TranslationStandardAxis=+Z  TranslationStandardOffset=0  TranslationStandardOffsetUnits=m  TranslationROffset=0  TranslationROffsetUnits=m  TranslationThetaOffset=0  TranslationThetaOffsetUnits=deg  TranslationZOffset=0  TranslationZOffsetUnits=m
  H : PMIOPort  Side=Left
  I : PMIOPort  Port=2  Side=Right
  connections:
  Black/RConn1 -- PlacIementI/LConn1 -- PlacementBlack/RConn1
  PlacementBlack/LConn1 -- H/RConn1
  I/RConn1 -- PlacIementI/RConn1

== system Simscape_model_Energy/ReferenceGenerator/Blue ==
  BlueBeam : sm_lib/Body Elements/Brick Solid  BrickDimensions=[LB2 w w]  BrickDimensionsUnits=m  ExportEntireGeometry=off  InertiaType=CalculateFromGeometry  BasedOnType=Mass  Density=0  DensityUnits=kg/m^3  Mass=0  MassUnits=kg  CenterOfMass=[0 0 0]  CenterOfMassUnits=m  MomentsOfInertia=[1 1 1]  MomentsOfInertiaUnits=kg*m^2  ProductsOfInertia=[0 0 0]  ProductsOfInertiaUnits=kg*m^2  GraphicType=FromGeometry  MarkerShape=Sphere  MarkerSize=10  GraphicVisPropType=SimpleVisualProperties  GraphicDiffuseColor=[0 0 1]  GraphicOpacity=1  GraphicSpecularColor=[0.5 0.5 0.5 1.0]  GraphicAmbientColor=[0.15 0.15 0.15 1.0]  GraphicEmissiveColor=[0.0 0.0 0.0 1.0]  GraphicShininess=75  DoExposeReferenceFrame=on  SerializedFrames=<Frames/>
  BlueBlock : sm_lib/Body Elements/Brick Solid  BrickDimensions=[LB1 LB3*2 LB3*2]  BrickDimensionsUnits=m  ExportEntireGeometry=off  InertiaType=Custom  BasedOnType=Mass  Density=1000  DensityUnits=kg/m^3  Mass=blueBlock.m  MassUnits=kg  CenterOfMass=[0 0 0]  CenterOfMassUnits=m  MomentsOfInertia=[blueBlock.Ix blueBlock.Iy blueBlock.Iz]  MomentsOfInertiaUnits=kg*m^2  ProductsOfInertia=[0 0 0]  ProductsOfInertiaUnits=kg*m^2  GraphicType=FromGeometry  MarkerShape=Sphere  MarkerSize=10  GraphicVisPropType=SimpleVisualProperties  GraphicDiffuseColor=[0 0 1]  GraphicOpacity=1  GraphicSpecularColor=[0.5 0.5 0.5 1.0]  GraphicAmbientColor=[0.15 0.15 0.15 1.0]  GraphicEmissiveColor=[0.0 0.0 0.0 1.0]  GraphicShininess=75  DoExposeReferenceFrame=on  SerializedFrames=<Frames/>
  PlacementB1 : sm_lib/Frames and Transforms/Rigid Transform  RotationMethod=RotationSequence  FollAlignAxisA=+X  BaseAlignAxisA=+Y  FollAlignAxisB=+Y  BaseAlignAxisB=+Z  RotationStandardAxis=+Z  RotationAngle=0  RotationAngleUnits=deg  RotationArbitraryAxis=[0 0 1]  RotationSequenceAxes=FollowerAxes  RotationSequence=XYX  RotationSequenceAngles=[90 0 0]  RotationSequenceAnglesUnits=deg  RotationMatrix=[1 0 0;0 1 0;0 0 1]  Quaternion=[1 0 0 0]  TranslationMethod=Cartesian  TranslationCartesianOffset=[LB3 0 LB1]  TranslationCartesianOffsetUnits=m  TranslationStandardAxis=+Z  TranslationStandardOffset=0  TranslationStandardOffsetUnits=m  TranslationROffset=0  TranslationROffsetUnits=m  TranslationThetaOffset=0  TranslationThetaOffsetUnits=deg  TranslationZOffset=0  TranslationZOffsetUnits=m
  PlacementBlueBeam : sm_lib/Frames and Transforms/Rigid Transform  RotationMethod=RotationSequence  FollAlignAxisA=+X  BaseAlignAxisA=+Y  FollAlignAxisB=+Y  BaseAlignAxisB=+Z  RotationStandardAxis=+Z  RotationAngle=0  RotationAngleUnits=deg  RotationArbitraryAxis=[0 0 1]  RotationSequenceAxes=FollowerAxes  RotationSequence=XYX  RotationSequenceAngles=[0 90 0]  RotationSequenceAnglesUnits=deg  RotationMatrix=[1 0 0;0 1 0;0 0 1]  Quaternion=[1 0 0 0]  TranslationMethod=Cartesian  TranslationCartesianOffset=[-LB1-LB2/2 0 LB3]  TranslationCartesianOffsetUnits=m  TranslationStandardAxis=+Z  TranslationStandardOffset=0  TranslationStandardOffsetUnits=m  TranslationROffset=0  TranslationROffsetUnits=m  TranslationThetaOffset=0  TranslationThetaOffsetUnits=deg  TranslationZOffset=0  TranslationZOffsetUnits=m
  PlacementBlueBlock : sm_lib/Frames and Transforms/Rigid Transform  RotationMethod=RotationSequence  FollAlignAxisA=+X  BaseAlignAxisA=+Y  FollAlignAxisB=+Y  BaseAlignAxisB=+Z  RotationStandardAxis=+Z  RotationAngle=0  RotationAngleUnits=deg  RotationArbitraryAxis=[0 0 1]  RotationSequenceAxes=FollowerAxes  RotationSequence=XYX  RotationSequenceAngles=[0 -90 0]  RotationSequenceAnglesUnits=deg  RotationMatrix=[1 0 0;0 1 0;0 0 1]  Quaternion=[1 0 0 0]  TranslationMethod=Cartesian  TranslationCartesianOffset=[LB1/2 0 0]  TranslationCartesianOffsetUnits=m  TranslationStandardAxis=+Z  TranslationStandardOffset=0  TranslationStandardOffsetUnits=m  TranslationROffset=0  TranslationROffsetUnits=m  TranslationThetaOffset=0  TranslationThetaOffsetUnits=deg  TranslationZOffset=0  TranslationZOffsetUnits=m
  SpringPlacement : sm_lib/Frames and Transforms/Rigid Transform  RotationMethod=None  FollAlignAxisA=+X  BaseAlignAxisA=+Y  FollAlignAxisB=+Y  BaseAlignAxisB=+Z  RotationStandardAxis=+Z  RotationAngle=0  RotationAngleUnits=deg  RotationArbitraryAxis=[0 0 1]  RotationSequenceAxes=FollowerAxes  RotationSequence=XYX  RotationSequenceAngles=[0 0 0]  RotationSequenceAnglesUnits=deg  RotationMatrix=[1 0 0;0 1 0;0 0 1]  Quaternion=[1 0 0 0]  TranslationMethod=Cartesian  TranslationCartesianOffset=[-LB2/2 0 0]  TranslationCartesianOffsetUnits=m  TranslationStandardAxis=+Z  TranslationStandardOffset=0  TranslationStandardOffsetUnits=m  TranslationROffset=0  TranslationROffsetUnits=m  TranslationThetaOffset=0  TranslationThetaOffsetUnits=deg  TranslationZOffset=0  TranslationZOffsetUnits=m
  A : PMIOPort  Side=Right
  B1 : PMIOPort  Port=2  Side=Right
  C : PMIOPort  Port=3  Side=Right
  connections:
  BlueBeam/RConn1 -- SpringPlacement/RConn1 -- PlacementBlueBeam/LConn1
  C/RConn1 -- SpringPlacement/LConn1
  BlueBlock/RConn1 -- PlacementBlueBlock/LConn1
  A/RConn1 -- PlacementB1/LConn1 -- PlacementBlueBlock/RConn1 -- PlacementBlueBeam/RConn1
  B1/RConn1 -- PlacementB1/RConn1
